simulink model "robc_mmc_simult_ccc"  (R2024b)
settings: Solver=FixedStepAuto  StartTime=0.0  StopTime=TSim  FixedStep=Ts  RelTol=1e-3
InitFcn:
  | load('fbg_c_controller_parameters.mat')
  | load('fb_c_controller_parameters.mat')
  | load('ff_c_controller_parameters.mat')
  | load('ss_c_model_parameters.mat')
  | load('operating_point_c_parameters.mat')
  | integralFlag = 0;
values from neighbouring files (symbols this model uses):
  Id_ref = 0    [main_simk_ccc.m]    (also in main_simk_occ.m = 1; main_simk_s.m = 1; operating_point_c_parameters.mat; operating_point_parameters.mat = 1)
  Iq_ref = 0    [main_simk_ccc.m]    (also in main_simk_occ.m; main_simk_s.m; operating_point_c_parameters.mat; operating_point_parameters.mat)
  Ts = 5e-05    [LoadParameters_SFC2K.mat]    (also in fb_c_controller_parameters.mat; fb_controller_parameters.mat; fbg_c_controller_parameters.mat; fbg_controller_parameters.mat)
  ulim = 1.2    [main_simk_ccc.m]    (also in main_simk_occ.m; main_simk_s.m; operating_point_c_parameters.mat; operating_point_parameters.mat)
  Vd_ = 0    [main_simk_ccc.m]    (also in main_simk_occ.m; main_simk_s.m; operating_point_c_parameters.mat; operating_point_parameters.mat)
  Vq_ = 0    [main_simk_ccc.m]    (also in main_simk_occ.m; main_simk_s.m; operating_point_c_parameters.mat; operating_point_parameters.mat)
  x0 = [0.1,0.1]'    [main_simk_ccc.m]
undefined symbols (not defined in the file or in its folder): DiscIntNeverNeededParam
settings Model: Creator=rmrane  LastModifiedBy=vreyesdreke
settings OptimizationCC: DefaultParameterBehavior=Inlined  EnhancedBackFolding=on  PassReuseOutputArgsAs=Individual arguments  ZeroExternalMemoryAtStartup=off  ZeroInternalMemoryAtStartup=off  OptimizeBlockOrder=speed  DifferentSizesBufferReuse=on  OptimizationCustomize=off  EfficientTunableParamExpr=on
settings DebuggingCC: ParameterTunabilityLossMsg=error
settings SFSimCC: MATLABDynamicMemAlloc=off
settings RTWCC: Description=Embedded Coder  SystemTargetFile=ert.tlc  TemplateMakefile=ert_default_tmf
settings CodeAppCC: GenerateComments=off  IgnoreCustomStorageClasses=off  OperatorAnnotations=on  SimulinkDataObjDesc=on  SFDataObjDesc=on  CustomSymbolStrType=$N$R$M  SimulinkBlockComments=off  InternalIdentifier=Classic
settings ERTTargetCC: GenerateSampleERTMain=on  SupportAbsoluteTime=off  SupportNonFinite=off  SupportComplex=off  ERTCustomFileTemplate=example_file_process.tlc  ConvertIfToSwitch=off  SuppressUnreachableDefaultCases=off  EnableSignedLeftShifts=off  EnableSignedRightShifts=off  DynamicArrayContainerType=coder::array

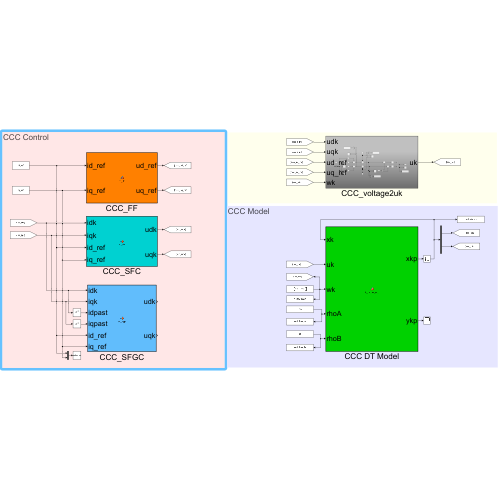
[thumbnail: Simulink's stored preview of the top-level diagram]
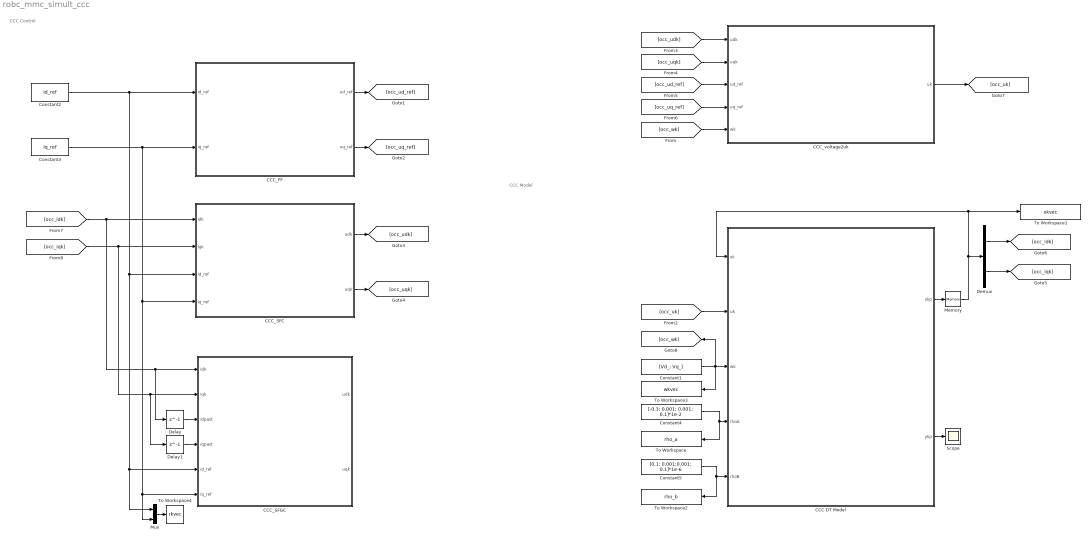
== system robc_mmc_simult_ccc ==
  note: CCC Model
  note: CCC Control
  CCC DT Model : MATLAB Function  TreatAsAtomicUnit=on
  CCC_FF : MATLAB Function  TreatAsAtomicUnit=on
  CCC_SFC : MATLAB Function  TreatAsAtomicUnit=on
  CCC_SFGC : MATLAB Function  TreatAsAtomicUnit=on
  CCC_voltage2uk : Subsystem
  Constant1 : Constant  Value=[Vd_; Vq_]  SampleTime=Ts
  Constant2 : Constant  Value=Id_ref  SampleTime=Ts
  Constant3 : Constant  Value=Iq_ref  SampleTime=Ts
  Constant4 : Constant  Value=[-0.3; 0.001; 0.001; 0.1]*1e-2  SampleTime=Ts
  Constant5 : Constant  Value=[0.1; 0.001;0.001; 0.1]*1e-6  SampleTime=Ts
  Delay : Delay  DelayLength=1  InputProcessing=Columns as channels (frame based)  SampleTime=Ts
  Delay1 : Delay  DelayLength=1  InputProcessing=Columns as channels (frame based)  SampleTime=Ts
  Demux : Demux  Outputs=2
  Memory : Memory  InitialCondition=x0  InheritSampleTime=on  LinearizeAsDelay=on
  Mux : Mux  Inputs=2
  Scope : Scope
  To Workspace : ToWorkspace  VariableName=rho_a  SampleTime=Ts
      settings: Save2DSignal=2-D array (concatenate along first dimension)
  To Workspace1 : ToWorkspace  VariableName=xkvec  SampleTime=Ts
      settings: Save2DSignal=2-D array (concatenate along first dimension)
  To Workspace2 : ToWorkspace  VariableName=rho_b  SampleTime=Ts
      settings: Save2DSignal=2-D array (concatenate along first dimension)
  To Workspace3 : ToWorkspace  VariableName=wkvec  SampleTime=Ts
      settings: Save2DSignal=2-D array (concatenate along first dimension)
  To Workspace4 : ToWorkspace  VariableName=rkvec  SampleTime=Ts
      settings: Save2DSignal=2-D array (concatenate along first dimension)
  wires:
  Constant1/1 -> [occ_wk], To Workspace3/1, CCC DT Model/3(wk)
  CCC DT Model/1(xkp) -> Memory/1
  CCC_FF/1(ud_ref) -> [occ_ud_ref]
  CCC_FF/2(uq_ref) -> [occ_uq_ref]
  Constant2/1 -> CCC_FF/1(id_ref), CCC_SFGC/5(id_ref), Mux/1, CCC_SFC/3(id_ref)
  Constant3/1 -> CCC_FF/2(iq_ref), Mux/2, CCC_SFGC/6(iq_ref), CCC_SFC/4(iq_ref)
  Memory/1 -> Demux/1, To Workspace1/1, CCC DT Model/1(xk)
  Demux/2 -> [occ_iqk]
  Demux/1 -> [occ_idk]
  CCC_voltage2uk/1(uk) -> [occ_uk]
  [occ_uk] -> CCC DT Model/2(uk)
  [occ_udk] -> CCC_voltage2uk/1(udk)
  [occ_uqk] -> CCC_voltage2uk/2(uqk)
  [occ_ud_ref] -> CCC_voltage2uk/3(ud_ref)
  [occ_uq_ref] -> CCC_voltage2uk/4(uq_ref)
  [occ_idk] -> Delay/1, CCC_SFGC/1(idk), CCC_SFC/1(idk)
  [occ_iqk] -> Delay1/1, CCC_SFGC/2(iqk), CCC_SFC/2(iqk)
  Constant4/1 -> To Workspace/1, CCC DT Model/4(rhoA)
  Constant5/1 -> To Workspace2/1, CCC DT Model/5(rhoB)
  CCC DT Model/2(ykp) -> Scope/1
  Delay/1 -> CCC_SFGC/3(idpast)
  Delay1/1 -> CCC_SFGC/4(iqpast)
  CCC_SFC/2(uqk) -> [occ_uqk]
  CCC_SFC/1(udk) -> [occ_udk]
  Mux/1 -> To Workspace4/1
  [occ_wk] -> CCC_voltage2uk/5(wk)

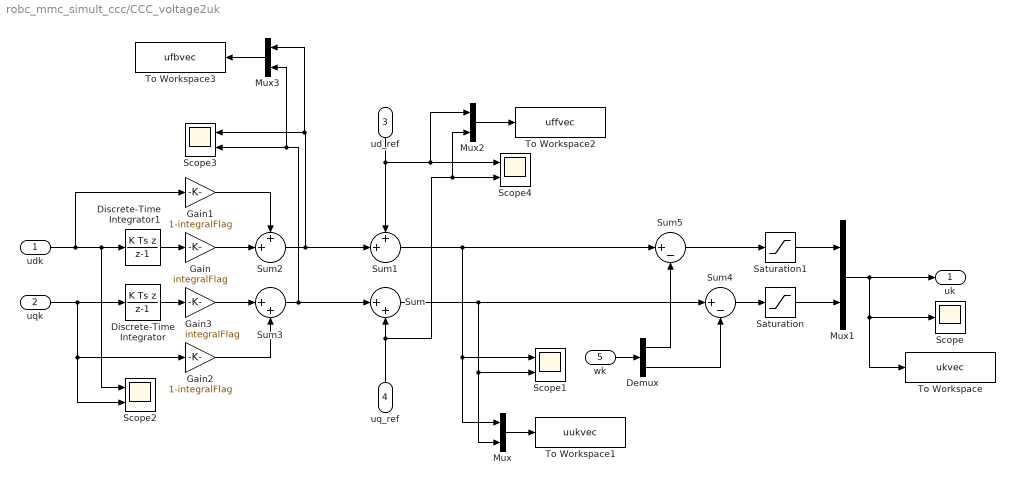
== system robc_mmc_simult_ccc/CCC_voltage2uk ==
  udk : Inport
  uqk : Inport  Port=2
  ud_ref : Inport  Port=3
  uq_ref : Inport  Port=4
  wk : Inport  Port=5
  Demux : Demux  Outputs=2
  Discrete-Time Integrator : DiscreteIntegrator  IntegratorMethod=Integration: Backward Euler  gainval=1.0/Ts  SampleTime=Ts  ICPrevOutput=DiscIntNeverNeededParam  ICPrevScaledInput=DiscIntNeverNeededParam
  Discrete-Time Integrator1 : DiscreteIntegrator  IntegratorMethod=Integration: Backward Euler  gainval=1.0/Ts  SampleTime=Ts  ICPrevOutput=DiscIntNeverNeededParam  ICPrevScaledInput=DiscIntNeverNeededParam
  Gain : Gain  Gain=integralFlag
  Gain1 : Gain  Gain=1-integralFlag
  Gain2 : Gain  Gain=1-integralFlag
  Gain3 : Gain  Gain=integralFlag
  Mux{,1..3} (4 alike) : Mux  Inputs=2
  Saturation : Saturate  UpperLimit=ulim  LowerLimit=-ulim
  Saturation1 : Saturate  UpperLimit=ulim  LowerLimit=-ulim
  Scope : Scope
  Scope{1..4} (4 alike) : Scope  NumInputPorts=2
  Sum : Sum  Inputs=|++
  Sum1 : Sum  Inputs=++|
  Sum2 : Sum  Inputs=++|
  Sum3 : Sum  Inputs=|++
  Sum4 : Sum  Inputs=|+-
  Sum5 : Sum  Inputs=|+-
  To Workspace : ToWorkspace  VariableName=ukvec  SampleTime=Ts
      settings: Save2DSignal=2-D array (concatenate along first dimension)
  To Workspace1 : ToWorkspace  VariableName=uukvec  SampleTime=Ts
      settings: Save2DSignal=2-D array (concatenate along first dimension)
  To Workspace2 : ToWorkspace  VariableName=uffvec  SampleTime=Ts
      settings: Save2DSignal=2-D array (concatenate along first dimension)
  To Workspace3 : ToWorkspace  VariableName=ufbvec  SampleTime=Ts
      settings: Save2DSignal=2-D array (concatenate along first dimension)
  uk : Outport
  wires:
  Sum2/1 -> Mux3/1, Scope3/1, Sum1/2
  Gain2/1 -> Sum3/2
  uq_ref/1 -> Mux2/2, Scope4/2, Sum/2
  ud_ref/1 -> Mux2/1, Scope4/1, Sum1/1
  udk/1 -> Scope2/1, Discrete-Time Integrator1/1, Gain1/1
  Discrete-Time Integrator1/1 -> Gain/1
  Sum/1 -> Sum4/1, Mux/2, Scope1/2
  Sum3/1 -> Mux3/2, Scope3/2, Sum/1
  Saturation/1 -> Mux1/2
  Mux1/1 -> To Workspace/1, Scope/1, uk/1
  Gain/1 -> Sum2/2
  Gain3/1 -> Sum3/1
  Saturation1/1 -> Mux1/1
  Sum1/1 -> Sum5/1, Mux/1, Scope1/1
  Discrete-Time Integrator/1 -> Gain3/1
  uqk/1 -> Scope2/2, Gain2/1, Discrete-Time Integrator/1
  Gain1/1 -> Sum2/1
  Mux/1 -> To Workspace1/1
  Mux2/1 -> To Workspace2/1
  Mux3/1 -> To Workspace3/1
  wk/1 -> Demux/1
  Demux/2 -> Sum4/2
  Demux/1 -> Sum5/2
  Sum5/1 -> Saturation1/1
  Sum4/1 -> Saturation/1

== matlab function robc_mmc_simult_ccc/CCC DT Model ==
  settings: updateMethod=DISCRETE  sampleTime=Ts
  data: xk input size=2; xkp output size=2; uk input size=2; ykp output size=2; wk input size=2; rhoA input size=4; rhoB input size=4
function [xkp,ykp] = dt_model_occ(xk, uk, wk, rhoA, rhoB)
% dt_model_occ(xk, uk, wk) discrete-time model of the MMC OCC dynamics.
    m_ss = coder.load('ss_c_model_parameters.mat','-mat','-regexp',...
        'A','B','C','D','E');
    dA = [rhoA(1), rhoA(2); rhoA(3), rhoA(4)];
    dB = [rhoB(1), rhoB(2); rhoB(3), rhoB(4)];
    xkp = (m_ss.A+dA)*xk+(m_ss.B+dB)*uk+m_ss.E*wk;
    ykp = m_ss.C*xk;
end

== matlab function robc_mmc_simult_ccc/CCC_SFC ==
  settings: updateMethod=DISCRETE  sampleTime=Ts
  data: idk input size=1; udk output size=1; iqk input size=1; uqk output size=1; id_ref input; iq_ref input
function [udk,uqk] = cc_sfc(idk, iqk,id_ref,iq_ref)
    % oc_sfc(idk, iqk,id_ref,iq_ref) feedforward controller gain.
    m_ss = coder.load('fb_c_controller_parameters.mat','-mat','-regexp','Kfb');
    uk = m_ss.Kfb*([idk, iqk]'-[id_ref,iq_ref]');
    udk = uk(1);
    uqk = uk(2);
end

== matlab function robc_mmc_simult_ccc/CCC_FF ==
  settings: updateMethod=DISCRETE  sampleTime=Ts
  data: id_ref input size=1; ud_ref output size=1; iq_ref input size=1; uq_ref output size=1
function [ud_ref,uq_ref] = cc_ffc(id_ref,iq_ref)
    % oc_ffc(id_ref,iq_ref) feedforward controller gain.
    m_ss = coder.load('ff_c_controller_parameters.mat','-mat','-regexp','Kff');
    uss = m_ss.Kff*[id_ref,iq_ref]';
    ud_ref = uss(1);
    uq_ref = uss(2);
end

== matlab function robc_mmc_simult_ccc/CCC_SFGC ==
  settings: updateMethod=DISCRETE  sampleTime=Ts
  data: idk input size=1; udk output size=1; iqk input size=1; idpast input size=1; iqpast input size=1; uqk output size=1; id_ref input; iq_ref input
function [udk,uqk] = cc_sfgc(idk, iqk,idpast, iqpast,id_ref,iq_ref)
    % oc_sfc(idk, iqk,id_ref,iq_ref) feedforward controller gain.
    m_ss = coder.load('fbg_c_controller_parameters.mat','-mat','-regexp','Kfbg');
    ekvec = [(idk-idpast), (iqk-iqpast),idk,iqk]'-[0,0,id_ref,iq_ref]';
    uk = m_ss.Kfbg*ekvec;
    udk = uk(1);
    uqk = uk(2);
end
